simulink model "Aerodynamic_Model"  (R2024a)
settings: Solver=FixedStepDiscrete  StartTime=0.0  StopTime=0  FixedStep=0.001  RelTol=1e-3
settings Model: Creator=zz  LastModifiedBy=zz

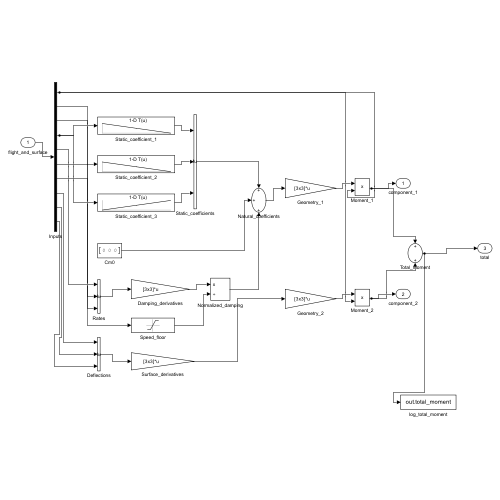
[thumbnail: Simulink's stored preview of the top-level diagram]
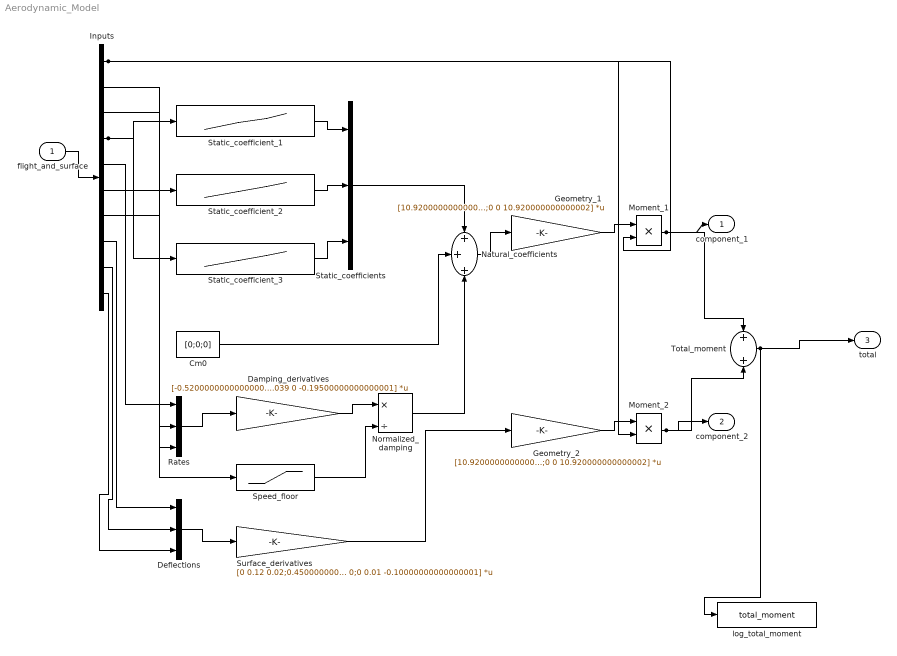
== system Aerodynamic_Model ==
  flight_and_surface : Inport  PortDimensions=10
  Cm0 : Constant  Value=[0;0;0]
  Damping_derivatives : Gain  Gain=[-0.52000000000000002 0 0.13;0 -19.200000000000003 0;-0.039 0 -0.19500000000000001]  Multiplication=Matrix(K*u)
  Deflections : Mux  Inputs=3
  Geometry_1 : Gain  Gain=[10.920000000000002 0 0;0 13.440000000000001 0;0 0 10.920000000000002]  Multiplication=Matrix(K*u)
  Geometry_2 : Gain  Gain=[10.920000000000002 0 0;0 13.440000000000001 0;0 0 10.920000000000002]  Multiplication=Matrix(K*u)
  Inputs : Demux  Outputs=10
  Moment_1 : Product
  Moment_2 : Product
  Natural_coefficients : Sum  Inputs=+++
  Normalized_damping : Product  Inputs=*/
  Rates : Mux  Inputs=3
  Speed_floor : Saturate  UpperLimit=inf  LowerLimit=1
  Static_coefficient_1 : Lookup_n-D  NumberOfTableDimensions=1  BreakpointsForDimension1=[-pi 0 pi]  Table=[0.25132741228718347 0 -0.25132741228718347]
  Static_coefficient_2 : Lookup_n-D  NumberOfTableDimensions=1  BreakpointsForDimension1=[-pi 0 pi]  Table=[1.0995574287564276 0 -1.0995574287564276]
  Static_coefficient_3 : Lookup_n-D  NumberOfTableDimensions=1  BreakpointsForDimension1=[-pi 0 pi]  Table=[-0.37699111843077515 0 0.37699111843077515]
  Static_coefficients : Mux  Inputs=3
  Surface_derivatives : Gain  Gain=[0 0.12 0.02;0.45000000000000001 0 0;0 0.01 -0.10000000000000001]  Multiplication=Matrix(K*u)
  Total_moment : Sum
  log_total_moment : ToWorkspace  VariableName=total_moment  SaveFormat=Timeseries
  component_1 : Outport
  component_2 : Outport  Port=2
  total : Outport  Port=3
  wires:
  flight_and_surface/1 -> Inputs/1
  Inputs/4 -> Static_coefficient_1/1, Static_coefficient_3/1
  Inputs/3 -> Static_coefficient_2/1
  Static_coefficient_1/1 -> Static_coefficients/1
  Static_coefficient_2/1 -> Static_coefficients/2
  Static_coefficient_3/1 -> Static_coefficients/3
  Inputs/5 -> Rates/1
  Inputs/8 -> Deflections/1
  Inputs/6 -> Rates/2
  Inputs/9 -> Deflections/2
  Inputs/7 -> Rates/3
  Inputs/10 -> Deflections/3
  Rates/1 -> Damping_derivatives/1
  Inputs/2 -> Speed_floor/1
  Damping_derivatives/1 -> Normalized_damping/1
  Speed_floor/1 -> Normalized_damping/2
  Deflections/1 -> Surface_derivatives/1
  Static_coefficients/1 -> Natural_coefficients/1
  Cm0/1 -> Natural_coefficients/2
  Normalized_damping/1 -> Natural_coefficients/3
  Natural_coefficients/1 -> Geometry_1/1
  Geometry_1/1 -> Moment_1/1
  Inputs/1 -> Moment_1/2, Moment_2/2
  Moment_1/1 -> component_1/1, Total_moment/1
  Surface_derivatives/1 -> Geometry_2/1
  Geometry_2/1 -> Moment_2/1
  Moment_2/1 -> component_2/1, Total_moment/2
  Total_moment/1 -> total/1, log_total_moment/1
